simulink library "Yaw_Controller_Lib"  (R2025a)
settings: Solver=ode45  StartTime=0.0  StopTime=10.0  RelTol=1e-3  EnableMultiTasking=on
undefined symbols (not defined in the file): WT_Params
libraries: $bdroot x1
Description:
  | Copyright 2009-2025 The MathWorks, Inc. MathWorks, Inc.
settings Model: Creator=smiller  LastModifiedBy=smiller
settings SolverCC: AlgebraicLoopSolver=TrustRegion
settings DataIOCC: LimitDataPoints=on  SaveFormat=Array  SignalLoggingSaveFormat=ModelDataLogs  ReturnWorkspaceOutputs=off
settings OptimizationCC: ReuseModelBlockBuffer=off  ExpressionDepthLimit=2147483647.0  LifeSpan=inf
settings DebuggingCC: UnderspecifiedInitializationDetection=Classic  MergeDetectMultiDrivingBlocksExec=none  SolverPrmCheckMsg=warning  FcnCallInpInsideContextMsg=warning  UnconnectedInputMsg=warning  UnconnectedOutputMsg=warning  UnconnectedLineMsg=warning  AllowSymbolicDim=off  StateNameClashWarn=warning  PregeneratedLibrarySubsystemCodeDiagnostic=none  SFUnexpectedBacktrackingDiag=warning  SFNoUnconditionalDefaultTransitionDiag=warning  SFExecutionAtInitializationDiag=none  ArithmeticOperatorsInVariantConditions=warning
settings HardwareCC: ProdBitPerPointer=32.0  ProdBitPerSizeT=32.0  ProdBitPerPtrDiffT=32.0  ProdLargestAtomicFloat=None  ProdIntDivRoundTo=Undefined  ProdEndianess=Unspecified  ProdWordSize=32.0  ProdHWDeviceType=32-bit Generic
settings ModelReferenceCC: EnableRefExpFcnMdlSchedulingChecks=on  PropagateSignalLabelsOutOfModel=off
settings SFSimCC: SimUseLocalCustomCode=off  CustomCodeUndefinedFunction=UseInterfaceOnly
settings RTWCC: RTWUseLocalCustomCode=off  GPUComputeCapability=3.5  DLArmComputeVersion=19.05
settings CodeAppCC: StateflowObjectComments=on
settings GRTTargetCC: TargetLangStandard=C89/C90 (ANSI)  CombineOutputUpdateFcns=off  GRTInterface=on
settings ConfigComp: CovMetricSettings=dw  CovSaveCumulativeToWorkspaceVar=on  CovSaveSingleToWorkspaceVar=on  CovExternalEMLEnable=off  CovSFcnEnable=off

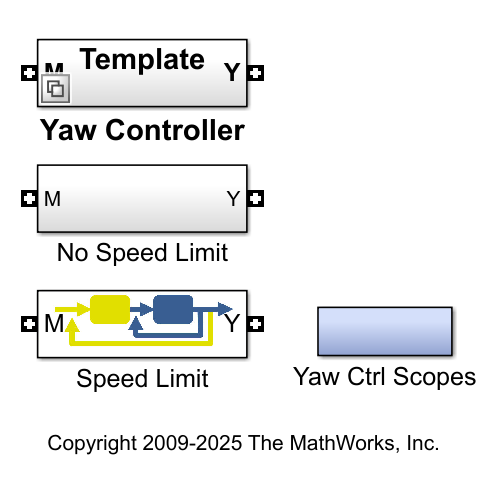
[thumbnail: Simulink's stored preview of the top-level diagram]
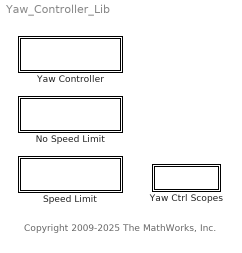
== system Yaw_Controller_Lib ==
  note: Copyright 2009-2025 The MathWorks, Inc.
  No Speed Limit : Subsystem
  Speed Limit : Subsystem
      mask Display:
      | image(imread('Yaw_Controller_Speed_Limit_IMAGE.jpg'));
      | port_label('LConn',1,'M');
      | port_label('RConn',1,'Y');
  Yaw Controller : Subsystem  BlockChoice=No Speed Limit
      settings: TemplateBlock=self  MemberBlocks=No Speed Limit,Speed Limit
  Yaw Ctrl Scopes : Subsystem

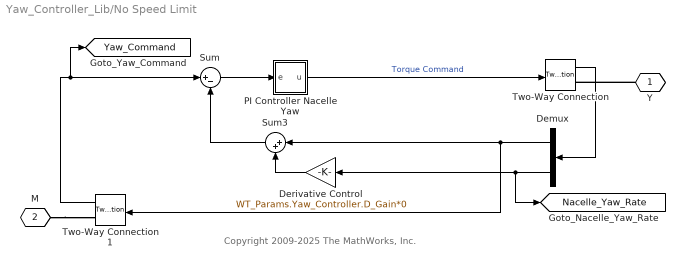
== system Yaw_Controller_Lib/No Speed Limit ==
  note: Copyright 2009-2025 The MathWorks, Inc.
  Demux : Demux  Outputs=[4 1]
  Derivative Control : Gain  Gain=WT_Params.Yaw_Controller.D_Gain*0
  PI Controller Nacelle Yaw : Subsystem  mask(PID Controller){P=WT_Params.Yaw_Controller.P_Gain, I=WT_Params.Yaw_Controller.I_Gain}
      mask prompts: P "Proportional:"; I "Integral:"
      mask help:
      | Enter expressions for proportional, integral, and derivative terms.
      | P+I/s+Ds
      mask Help: This block implements a PID controller where parameters are entered for the Proportional, Integral and Derivative terms. Unmask this block to see how it works. The derivative term is implemented using a true derivative block.
      mask Display: disp('PI')
  Sum : Sum  Inputs=|+-
  Sum3 : Sum  Inputs=|++
  Two-Way Connection : TwoWayConnection
  Two-Way Connection1 : TwoWayConnection
  Y : PMIOPort  Tag=PMCPort  Side=Right
  M : PMIOPort  Tag=PMCPort  Port=2  Side=Left
  tag scope: Nacelle_Yaw_Rate=global, Yaw_Command=global
  wires:
  Derivative Control/1 -> Sum3/2
  Sum3/1 -> Sum/2
  Two-Way Connection1/1 -> [Yaw_Command], Sum/1
  Two-Way Connection/1 -> Demux/1
  Demux/1 -> Sum3/1, Two-Way Connection1/1
  Sum/1 -> PI Controller Nacelle Yaw/1(e)
  PI Controller Nacelle Yaw/1(u) -> Two-Way Connection/1  "Torque Command"
  Demux/2 -> Derivative Control/1, [Nacelle_Yaw_Rate]
  connections:
  M/RConn1 -- Two-Way Connection1/RConn1
  Y/RConn1 -- Two-Way Connection/RConn1

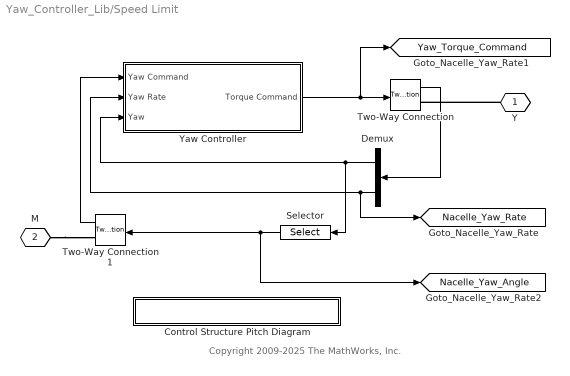
== system Yaw_Controller_Lib/Speed Limit ==
  note: Copyright 2009-2025 The MathWorks, Inc.
  Control Structure Pitch Diagram : Subsystem
      mask Display: disp('View Yaw Control Structure');
  Demux : Demux  Outputs=[4 1]
  Selector : Selector  InputPortWidth=4  IndexOptions=Index vector (dialog)  Indices=[1 ]  OutputSizes=1
  Two-Way Connection : TwoWayConnection
  Two-Way Connection1 : TwoWayConnection
  Yaw Controller : Subsystem
  Y : PMIOPort  Tag=PMCPort  Side=Right
  M : PMIOPort  Tag=PMCPort  Port=2  Side=Left
  tag scope: Nacelle_Yaw_Angle=global, Nacelle_Yaw_Rate=global, Yaw_Torque_Command=global
  wires:
  Yaw Controller/1(Torque Command) -> Two-Way Connection/1, [Yaw_Torque_Command]
  Two-Way Connection/1 -> Demux/1
  Demux/1 -> Yaw Controller/3(Yaw), Selector/1
  Demux/2 -> [Nacelle_Yaw_Rate], Yaw Controller/2(Yaw Rate)
  Two-Way Connection1/1 -> Yaw Controller/1(Yaw Command)
  Selector/1 -> Two-Way Connection1/1, [Nacelle_Yaw_Angle]
  connections:
  M/RConn1 -- Two-Way Connection1/RConn1
  Y/RConn1 -- Two-Way Connection/RConn1

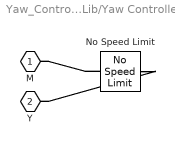
== system Yaw_Controller_Lib/Yaw Controller ==
  No Speed Limit : $bdroot/No Speed Limit  SystemSampleTime=-1  VariantActivationTime=update diagram  EmptyChoice=off  PassThrough=off  PassThroughVariantControl=(default)  EmptyChoiceVariantControl=(default)  AllowFlexibleInterface=on  Latency=0  AutoFrameSizeCalculation=off
  M : PMIOPort  Side=Left
  Y : PMIOPort  Port=2  Side=Right
  connections:
  No Speed Limit/LConn1 -- M/RConn1
  No Speed Limit/RConn1 -- Y/RConn1

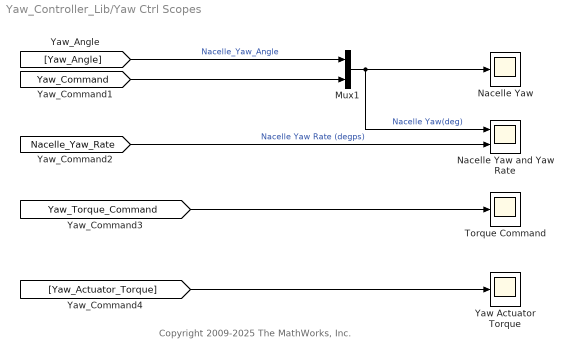
== system Yaw_Controller_Lib/Yaw Ctrl Scopes ==
  note: Copyright 2009-2025 The MathWorks, Inc.
  Mux1 : Mux  Inputs=2
  Nacelle Yaw : Scope
      settings: TimeSpan=80  DataLoggingVariableName=Nacelle_Yaw_DATA
  Nacelle Yaw and Yaw Rate : Scope  NumInputPorts=2
      settings: TimeSpan=80  ActiveDisplayYMinimum=-5  ActiveDisplayYMaximum=5  DataLoggingVariableName=ScopeData7
  Torque Command : Scope
      settings: TimeSpan=3.951473136915078
  Yaw Actuator Torque : Scope
      settings: TimeSpan=3.951473136915078  DataLoggingVariableName=Yaw_Actuator_Torque_DATA
  wires:
  [Yaw_Actuator_Torque] -> Yaw Actuator Torque/1
  [Yaw_Torque_Command] -> Torque Command/1
  [Yaw_Angle] -> Mux1/1  "Nacelle_Yaw_Angle"
  [Yaw_Command] -> Mux1/2
  Mux1/1 -> Nacelle Yaw and Yaw Rate/1, Nacelle Yaw/1  "Nacelle Yaw(deg)"
  [Nacelle_Yaw_Rate] -> Nacelle Yaw and Yaw Rate/2  "Nacelle Yaw Rate (degps)"

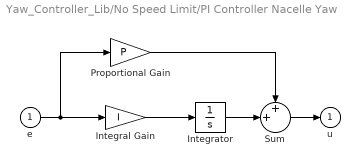
== system Yaw_Controller_Lib/No Speed Limit/PI Controller Nacelle Yaw ==
  e : Inport
  Integral Gain : Gain  Gain=I  SaturateOnIntegerOverflow=on  OutDataTypeStr=Inherit: Same as input  ParamDataTypeStr=Inherit: Same as input
  Integrator : Integrator
  Proportional Gain : Gain  Gain=P  SaturateOnIntegerOverflow=on  OutDataTypeStr=Inherit: Same as input  ParamDataTypeStr=Inherit: Same as input
  Sum : Sum  Inputs=++|  InputSameDT=on  SaturateOnIntegerOverflow=on  OutDataTypeStr=Inherit: Same as first input
  u : Outport  InitialOutput=0  VectorParamsAs1DForOutWhenUnconnected=off
  wires:
  Sum/1 -> u/1
  e/1 -> Integral Gain/1, Proportional Gain/1
  Integrator/1 -> Sum/2
  Proportional Gain/1 -> Sum/1
  Integral Gain/1 -> Integrator/1

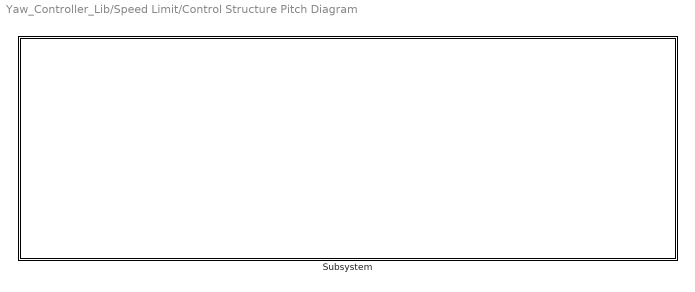
== system Yaw_Controller_Lib/Speed Limit/Control Structure Pitch Diagram ==
  Subsystem : Subsystem
      mask Display: image(imread('Control_Structure_Yaw_IMAGE.jpg'));

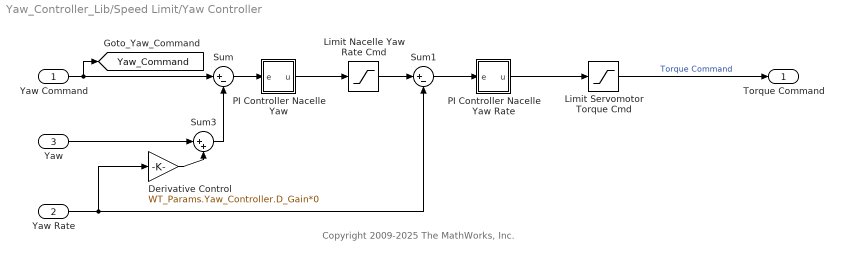
== system Yaw_Controller_Lib/Speed Limit/Yaw Controller ==
  note: Copyright 2009-2025 The MathWorks, Inc.
  Yaw Command : Inport
  Yaw Rate : Inport  Port=2
  Yaw : Inport  Port=3
  Derivative Control : Gain  Gain=WT_Params.Yaw_Controller.D_Gain*0
  Limit Nacelle Yaw Rate Cmd : Saturate  UpperLimit=WT_Params.Yaw_Actuator.max_yaw_rate  LowerLimit=-WT_Params.Yaw_Actuator.max_yaw_rate
  Limit Servomotor Torque Cmd : Saturate  UpperLimit=max(WT_Params.Yaw_Actuator.Motor.max_torque_vector)  LowerLimit=-max(WT_Params.Yaw_Actuator.Motor.max_torque_vector)
  PI Controller Nacelle Yaw : Subsystem
      mask Display:
      | plot([0 1],[0 0]);
      | plot([1 2],[0 1]);
      | plot([2 3],[1 1]);
      | disp('P I');
  PI Controller Nacelle Yaw Rate : Subsystem
      mask Display:
      | plot([0 1],[0 0]);
      | plot([1 2],[0 1]);
      | plot([2 3],[1 1]);
      | disp('P I');
  Sum : Sum  Inputs=|+-
  Sum1 : Sum  Inputs=|+-
  Sum3 : Sum  Inputs=|++
  Torque Command : Outport  VectorParamsAs1DForOutWhenUnconnected=off
  tag scope: Yaw_Command=global
  wires:
  PI Controller Nacelle Yaw Rate/1(u) -> Limit Servomotor Torque Cmd/1
  PI Controller Nacelle Yaw/1(u) -> Limit Nacelle Yaw Rate Cmd/1
  Sum1/1 -> PI Controller Nacelle Yaw Rate/1(e)
  Limit Nacelle Yaw Rate Cmd/1 -> Sum1/1
  Derivative Control/1 -> Sum3/2
  Sum3/1 -> Sum/2
  Yaw Command/1 -> [Yaw_Command], Sum/1
  Sum/1 -> PI Controller Nacelle Yaw/1(e)
  Yaw/1 -> Sum3/1
  Yaw Rate/1 -> Sum1/2, Derivative Control/1
  Limit Servomotor Torque Cmd/1 -> Torque Command/1  "Torque Command"

== system Yaw_Controller_Lib/Speed Limit/Control Structure Pitch Diagram/Subsystem ==

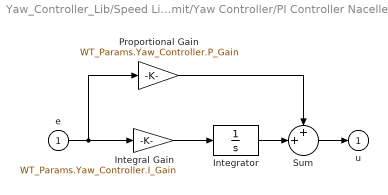
== system Yaw_Controller_Lib/Speed Limit/Yaw Controller/PI Controller Nacelle Yaw ==
  e : Inport
  Integral Gain : Gain  Gain=WT_Params.Yaw_Controller.I_Gain  SaturateOnIntegerOverflow=on  OutDataTypeStr=Inherit: Same as input  ParamDataTypeStr=Inherit: Same as input
  Integrator : Integrator  LimitOutput=on  UpperSaturationLimit=WT_Params.Yaw_Actuator.max_yaw_rate  LowerSaturationLimit=-WT_Params.Yaw_Actuator.max_yaw_rate
  Proportional Gain : Gain  Gain=WT_Params.Yaw_Controller.P_Gain  SaturateOnIntegerOverflow=on  OutDataTypeStr=Inherit: Same as input  ParamDataTypeStr=Inherit: Same as input
  Sum : Sum  Inputs=++|  InputSameDT=on  SaturateOnIntegerOverflow=on  OutDataTypeStr=Inherit: Same as first input
  u : Outport  InitialOutput=0  VectorParamsAs1DForOutWhenUnconnected=off
  wires:
  Sum/1 -> u/1
  e/1 -> Integral Gain/1, Proportional Gain/1
  Integrator/1 -> Sum/2
  Proportional Gain/1 -> Sum/1
  Integral Gain/1 -> Integrator/1

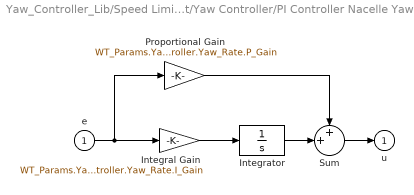
== system Yaw_Controller_Lib/Speed Limit/Yaw Controller/PI Controller Nacelle Yaw Rate ==
  e : Inport
  Integral Gain : Gain  Gain=WT_Params.Yaw_Controller.Yaw_Rate.I_Gain  SaturateOnIntegerOverflow=on  OutDataTypeStr=Inherit: Same as input  ParamDataTypeStr=Inherit: Same as input
  Integrator : Integrator  LimitOutput=on  UpperSaturationLimit=max(WT_Params.Yaw_Actuator.Motor.max_torque_vector)  LowerSaturationLimit=-max(WT_Params.Yaw_Actuator.Motor.max_torque_vector)
  Proportional Gain : Gain  Gain=WT_Params.Yaw_Controller.Yaw_Rate.P_Gain  SaturateOnIntegerOverflow=on  OutDataTypeStr=Inherit: Same as input  ParamDataTypeStr=Inherit: Same as input
  Sum : Sum  Inputs=++|  InputSameDT=on  SaturateOnIntegerOverflow=on  OutDataTypeStr=Inherit: Same as first input
  u : Outport  InitialOutput=0  VectorParamsAs1DForOutWhenUnconnected=off
  wires:
  Integral Gain/1 -> Integrator/1
  Proportional Gain/1 -> Sum/1
  Integrator/1 -> Sum/2
  e/1 -> Proportional Gain/1, Integral Gain/1
  Sum/1 -> u/1
